simulink library "lib_SecCtrl_Matrices"  (R2026a)
settings: Solver=VariableStepAuto
undefined symbols (not defined in the file): A_f_sc, A_P_sc, A_Q_sc, A_v_sc, buses_lf
settings Model: Creator=atomas  LastModifiedBy=atomas

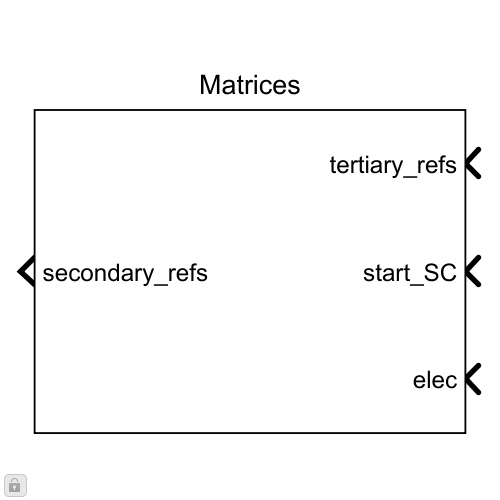
[thumbnail: Simulink's stored preview of the top-level diagram]
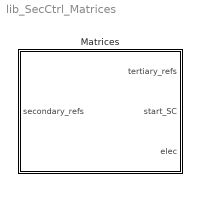
== system lib_SecCtrl_Matrices ==
  Matrices : Subsystem  VariantControl=Matrices

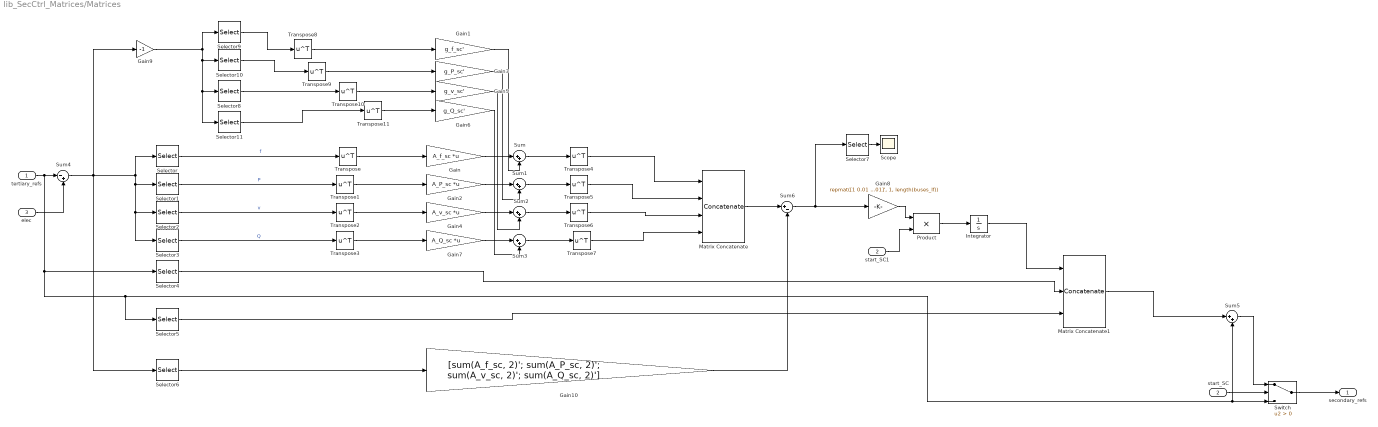
== system lib_SecCtrl_Matrices/Matrices ==
  tertiary_refs : Inport
  start_SC : Inport  Port=2
  elec : Inport  Port=3
  Gain : Gain  Gain=A_f_sc  Multiplication=Matrix(K*u)
  Gain1 : Gain  Gain=g_f_sc'
  Gain10 : Gain  Gain=[sum(A_f_sc, 2)'; sum(A_P_sc, 2)'; sum(A_v_sc, 2)'; sum(A_Q_sc, 2)']
  Gain2 : Gain  Gain=A_P_sc  Multiplication=Matrix(K*u)
  Gain3 : Gain  Gain=g_P_sc'
  Gain4 : Gain  Gain=A_v_sc  Multiplication=Matrix(K*u)
  Gain5 : Gain  Gain=g_v_sc'
  Gain6 : Gain  Gain=g_Q_sc'
  Gain7 : Gain  Gain=A_Q_sc  Multiplication=Matrix(K*u)
  Gain8 : Gain  Gain=repmat([1 0.01 1 0.01]', 1, length(buses_lf))
  Gain9 : Gain  Gain=-1
  Integrator : Integrator
  Matrix Concatenate : Concatenate  NumInputs=4  Mode=Multidimensional array
  Matrix Concatenate1 : Concatenate  NumInputs=3  Mode=Multidimensional array
  Product : Product
  Scope : Scope
      settings: ActiveDisplayYMinimum=-0.00016  ActiveDisplayYMaximum=0.00015
  Selector : Selector  NumberOfDimensions=2  InputPortWidth=3  IndexOptions=Index vector (dialog),Select all  Indices=1,1  OutputSizes=1,1
  Selector1 : Selector  NumberOfDimensions=2  InputPortWidth=3  IndexOptions=Index vector (dialog),Select all  Indices=2,1  OutputSizes=1,1
  Selector10 : Selector  NumberOfDimensions=2  InputPortWidth=3  IndexOptions=Index vector (dialog),Select all  Indices=2,1  OutputSizes=1,1
  Selector11 : Selector  NumberOfDimensions=2  InputPortWidth=3  IndexOptions=Index vector (dialog),Select all  Indices=4,1  OutputSizes=1,1
  Selector2 : Selector  NumberOfDimensions=2  InputPortWidth=3  IndexOptions=Index vector (dialog),Select all  Indices=3,1  OutputSizes=1,1
  Selector3 : Selector  NumberOfDimensions=2  InputPortWidth=3  IndexOptions=Index vector (dialog),Select all  Indices=4,1  OutputSizes=1,1
  Selector4 : Selector  NumberOfDimensions=2  InputPortWidth=3  IndexOptions=Index vector (dialog),Select all  Indices=5,1  OutputSizes=1,1
  Selector5 : Selector  NumberOfDimensions=2  InputPortWidth=3  IndexOptions=Index vector (dialog),Select all  Indices=6,1  OutputSizes=1,1
  Selector6 : Selector  NumberOfDimensions=2  InputPortWidth=3  IndexOptions=Index vector (dialog),Select all  Indices=1:4,1  OutputSizes=1,1
  Selector7 : Selector  NumberOfDimensions=2  InputPortWidth=3  IndexOptions=Index vector (dialog),Select all  Indices=1,1  OutputSizes=1,1
  Selector8 : Selector  NumberOfDimensions=2  InputPortWidth=3  IndexOptions=Index vector (dialog),Select all  Indices=3,1  OutputSizes=1,1
  Selector9 : Selector  NumberOfDimensions=2  InputPortWidth=3  IndexOptions=Index vector (dialog),Select all  Indices=1,1  OutputSizes=1,1
  Sum{,1..3,5} (5 alike) : Sum  Inputs=|++
  Sum4 : Sum  Inputs=|-+
  Sum6 : Sum  Inputs=|+-
  Switch : Switch  Criteria=u2 > Threshold  SaturateOnIntegerOverflow=off  InputSameDT=off
  Transpose{,1..11} (12 alike) : Math  Operator=transpose
  start_SC1 : InportShadow  Port=2
  secondary_refs : Outport
  wires:
  Gain10/1 -> Sum6/2
  start_SC1/1 -> Product/2
  Gain8/1 -> Product/1
  Selector7/1 -> Scope/1
  Sum6/1 -> Gain8/1, Selector7/1
  Product/1 -> Integrator/1
  Gain9/1 -> Selector9/1, Selector10/1, Selector8/1, Selector11/1
  Selector6/1 -> Gain10/1
  Matrix Concatenate/1 -> Sum6/1
  Integrator/1 -> Matrix Concatenate1/1
  Sum4/1 -> Selector/1, Selector1/1, Selector3/1, Selector2/1, Gain9/1, Selector6/1
  Transpose11/1 -> Gain6/1
  Transpose10/1 -> Gain5/1
  Transpose9/1 -> Gain3/1
  Transpose8/1 -> Gain1/1
  Sum5/1 -> Switch/1
  Matrix Concatenate1/1 -> Sum5/1
  Selector11/1 -> Transpose11/1
  Selector10/1 -> Transpose9/1
  Selector9/1 -> Transpose8/1
  Selector5/1 -> Matrix Concatenate1/3
  elec/1 -> Sum4/2
  Transpose5/1 -> Matrix Concatenate/2
  tertiary_refs/1 -> Sum4/1, Selector4/1, Selector5/1, Sum5/2, Switch/3
  Switch/1 -> secondary_refs/1
  start_SC/1 -> Switch/2
  Selector4/1 -> Matrix Concatenate1/2
  Selector8/1 -> Transpose10/1
  Transpose7/1 -> Matrix Concatenate/4
  Transpose6/1 -> Matrix Concatenate/3
  Transpose4/1 -> Matrix Concatenate/1
  Transpose3/1 -> Gain7/1
  Transpose2/1 -> Gain4/1
  Transpose1/1 -> Gain2/1
  Transpose/1 -> Gain/1
  Gain7/1 -> Sum3/1
  Sum3/1 -> Transpose7/1
  Sum2/1 -> Transpose6/1
  Gain6/1 -> Sum3/2
  Gain5/1 -> Sum2/2
  Gain4/1 -> Sum2/1
  Sum1/1 -> Transpose5/1
  Gain3/1 -> Sum1/2
  Gain2/1 -> Sum1/1
  Gain1/1 -> Sum/2
  Sum/1 -> Transpose4/1
  Gain/1 -> Sum/1
  Selector2/1 -> Transpose2/1  "v"
  Selector1/1 -> Transpose1/1  "P"
  Selector/1 -> Transpose/1  "f"
  Selector3/1 -> Transpose3/1  "Q"
